simulink model "sf_varsize_example"  (R2025b)
settings: Solver=FixedStepDiscrete  StartTime=0.0  StopTime=8  FixedStep=0.05  RelTol=1e-3  EnableMultiTasking=on
settings Model: Creator=The MathWorks, Inc.  LastModifiedBy=The MathWorks, Inc.
settings SolverCC: AlgebraicLoopSolver=TrustRegion
settings DataIOCC: LimitDataPoints=on  SaveFormat=Array  ReturnWorkspaceOutputs=off
settings OptimizationCC: ReuseModelBlockBuffer=off  ExpressionDepthLimit=2147483647.0  LifeSpan=inf
settings DebuggingCC: UnderspecifiedInitializationDetection=Classic  MergeDetectMultiDrivingBlocksExec=none  SolverPrmCheckMsg=warning  FcnCallInpInsideContextMsg=warning  UnconnectedInputMsg=warning  UnconnectedOutputMsg=warning  UnconnectedLineMsg=warning  StateNameClashWarn=warning  SFUnexpectedBacktrackingDiag=warning  SFNoUnconditionalDefaultTransitionDiag=warning  SFExecutionAtInitializationDiag=none  ArithmeticOperatorsInVariantConditions=warning
settings HardwareCC: ProdBitPerPointer=32.0  ProdBitPerSizeT=32.0  ProdBitPerPtrDiffT=32.0  ProdLargestAtomicFloat=None  ProdIntDivRoundTo=Undefined  ProdEndianess=Unspecified  ProdWordSize=32.0  ProdHWDeviceType=32-bit Generic
settings ModelReferenceCC: EnableRefExpFcnMdlSchedulingChecks=on  PropagateSignalLabelsOutOfModel=off
settings SFSimCC: SimUseLocalCustomCode=off  SimParseCustomCode=off  CustomCodeUndefinedFunction=UseInterfaceOnly
settings RTWCC: RTWUseLocalCustomCode=off  GPUComputeCapability=3.5  DLArmComputeVersion=19.05
settings CodeAppCC: StateflowObjectComments=on
settings GRTTargetCC: TargetLangStandard=C89/C90 (ANSI)  CombineOutputUpdateFcns=off  GRTInterface=on
settings ConfigComp: CovMetricSettings=dw  CovSaveCumulativeToWorkspaceVar=on  CovSaveSingleToWorkspaceVar=on  CovExternalEMLEnable=off  CovSFcnEnable=off

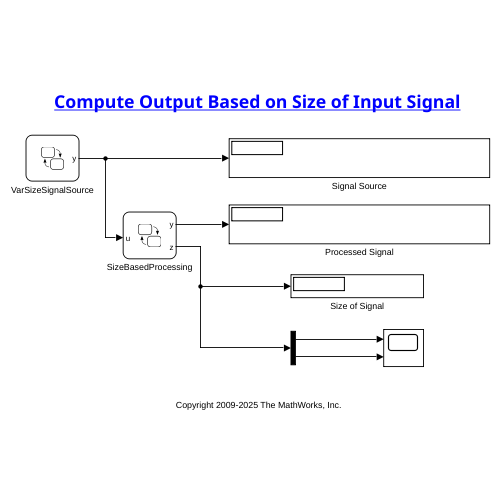
[thumbnail: Simulink's stored preview of the top-level diagram]
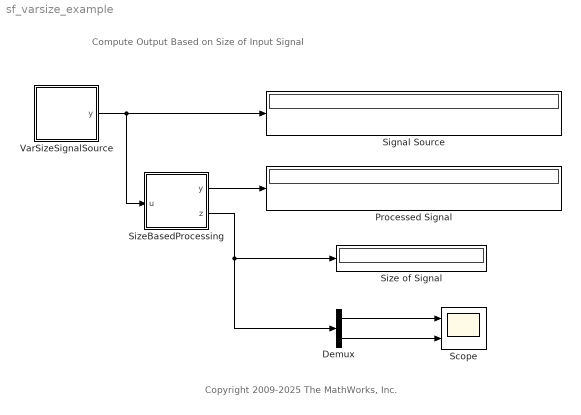
== system sf_varsize_example ==
  note: Copyright 2009-2025 The MathWorks, Inc.
  note: Compute Output Based on Size of Input Signal
  Demux : Demux  Outputs=2
  Processed Signal : Display
  Scope : Scope  NumInputPorts=2
      settings: Title=Columns  ActiveDisplayYMinimum=0.62500000000000011  ActiveDisplayYMaximum=4.375
  Signal Source : Display
  Size of Signal : Display
  SizeBasedProcessing : Stateflow chart  TreatAsAtomicUnit=on
  VarSizeSignalSource : Stateflow chart  TreatAsAtomicUnit=on
  wires:
  VarSizeSignalSource/1(y) -> SizeBasedProcessing/1(u), Signal Source/1
  SizeBasedProcessing/1(y) -> Processed Signal/1
  SizeBasedProcessing/2(z) -> Demux/1, Size of Signal/1
  Demux/1 -> Scope/1
  Demux/2 -> Scope/2

== stateflow chart sf_varsize_example/VarSizeSignalSource ==
  state Scalar
    en:
    y = 1;
  state Matrix
    en:
    y = reshape(1:8,[2 4]);
  state ColumnVector
    en:
    y = (1:2)';
  state RowVector
    en:
    y = (1:4);
  (default) -> Scalar
  Matrix -> Scalar : after(1,sec)
  Scalar -> ColumnVector : after(1,sec)
  RowVector -> Matrix : after(1,sec)
  ColumnVector -> RowVector : after(1,sec)
  data: y output double size=[2 4]

== stateflow chart sf_varsize_example/SizeBasedProcessing ==
  state Scalar
    computeOutput(0);
  state ColumnVector
    computeOutput(1);
  state RowVector
    computeOutput(2);
  state Matrix
    computeOutput(3);
  (default) -> (junction 42)
  (junction 47) -> (junction 42)
  (junction 42) -> (junction 38) : {readInputSize();}
  (junction 45) -> (junction 47)
  (junction 38) -> Scalar [order 1] : [z[0] == 1 && z[1] == 1]
  Scalar -> (junction 45)
  (junction 38) -> (junction 52) [order 2]
  (junction 62) -> (junction 45)
  (junction 52) -> ColumnVector [order 1] : [z[1] == 1]
  ColumnVector -> (junction 62)
  (junction 52) -> (junction 55) [order 2]
  (junction 65) -> (junction 62)
  (junction 55) -> RowVector [order 1] : [z[0] == 1]
  RowVector -> (junction 65)
  (junction 55) -> (junction 58) [order 2]
  (junction 68) -> (junction 65)
  (junction 58) -> Matrix
  Matrix -> (junction 68)
  data: key function_input double; u input double; y output double size=[2 4]; z output double size=[1 2]
  function readInputSize:
    | function readInputSize
    | %#codegen
    | z = size(u);
    | end
  function computeOutput(key):
    | function computeOutput(key)
    | %#codegen
    | switch key
    |     case 0 % scalar
    |         y = 0;
    |     case 1 % column vector
    |         y = sin(u);
    |     case 2 % row vector
    |         y = cos(u);
    |     case 3 % matrix
    |         y = sqrt(u);
    | end
    | end
